simulink model "SlidingModeObserverTest"  (R2026b)
settings: Solver=FixedStepDiscrete  StopTime=smoTestCfg.Duration  FixedStep=smoCfg.Ts
PostLoadFcn:
  | addpath(fullfile(fileparts(get_param(bdroot,'FileName')),'..','build_process'));initialize_smo_test(bdroot);
model workspace (MAT data in the model file):
  pllCfg.Ts = 5e-05
  pllCfg.NaturalFrequency = 40
  pllCfg.Damping = 0.707
  pllCfg.Kp = 355.376960974
  pllCfg.Ki = 63165.468167
  pllCfg.Kaw = 502.654824574
  pllCfg.OmegaMax = 1500
  pllCfg.MinMagnitude = 1
  pllCfg.LockError = 0.12
  pllCfg.LockSamples = 100
  pllCfg.Theta0 = 0
  pllCfg.Omega0 = 0
  smoCfg.Ts = 5e-05
  smoCfg.Rs = 0.5
  smoCfg.L = 0.001
  smoCfg.Flux = 0.035
  smoCfg.PolePairs = 4
  smoCfg.SlidingGain = 30
  smoCfg.Boundary = 1
  smoCfg.FilterHz = 600
  smoCfg.MinEmf = 1
  smoCfg.MinOmega = 30
  smoCfg.Compensate = 1
  smoCfg.A = 0.975309912028
  smoCfg.B = 0.0493801759433
  smoCfg.FilterA = 0.828204181307
  smoCfg.BoundaryPole = -0.506095366272
  smoTestCfg.Duration = 0.3
  smoTestCfg.ElectricalSpeed = 200
  smoTestCfg.InitialAngle = 0.4
  smoTestCfg.Iq = 2
  testStim.time = [0 5e-05 0.0001 0.00015 0.0002 0.00025 0.0003 0.00035 0.0004 0.00045 0.0005 0.00055 ... (6001 elements, 6001x1)]
  testStim.signals.values = [-3.48377113607 -3.555722953 -3.6273192006 -3.6985527193 -3.76941638582 -3.83990311383 -3.91000585473 -3.97971759831 -4.04903137344 -4.11794024881 -4.18643733359 -4.25451577812 ... (54009 elements, 6001x9)]
  testStim.signals.dimensions = 9
libraries: SlidingModeObserver x1
settings Model: Creator=24322  LastModifiedBy=24322

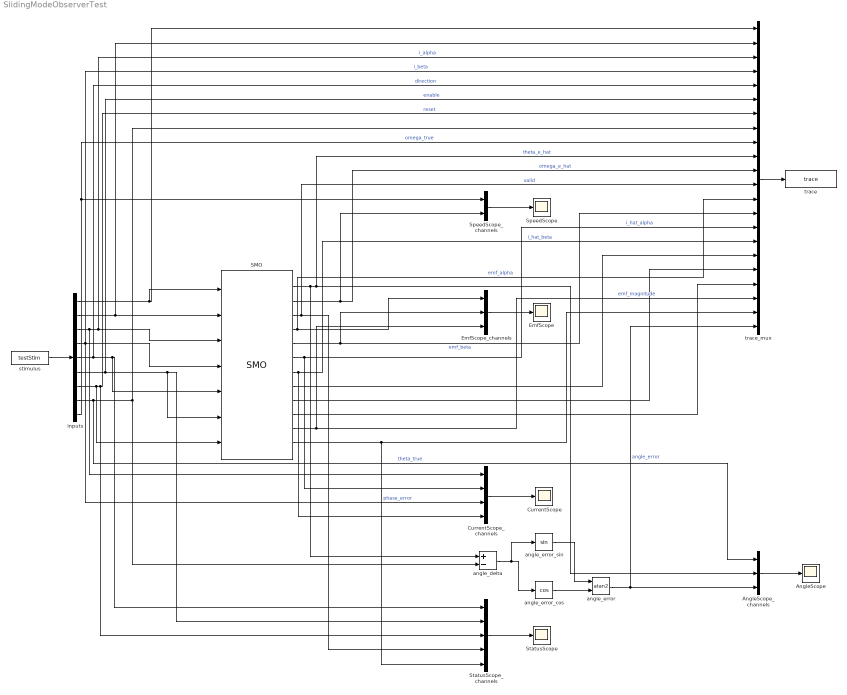
== system SlidingModeObserverTest ==
  AngleScope : Scope
  AngleScope_channels : Mux  Inputs=3
  CurrentScope : Scope
  CurrentScope_channels : Mux
  EmfScope : Scope
  EmfScope_channels : Mux  Inputs=3
  SMO : SlidingModeObserver/SMO  SystemSampleTime=-1  VariantActivationTime=update diagram  EmptyChoice=off  PassThrough=off  PassThroughVariantControl=(default)  EmptyChoiceVariantControl=(default)  AllowFlexibleInterface=on  Latency=0  AutoFrameSizeCalculation=off
  SpeedScope : Scope
  SpeedScope_channels : Mux  Inputs=2
  StatusScope : Scope
  StatusScope_channels : Mux  Inputs=5
  angle_delta : Sum  Inputs=+-
  angle_error : Trigonometry  Operator=atan2
  angle_error_cos : Trigonometry  Operator=cos
  angle_error_sin : Trigonometry
  inputs : Demux  Outputs=9
  stimulus : FromWorkspace  VariableName=testStim  SampleTime=smoCfg.Ts  Interpolate=off  OutputAfterFinalValue=Holding final value
  trace : ToWorkspace  VariableName=trace  SaveFormat=Structure With Time  SampleTime=-1
  trace_mux : Mux  Inputs=22
  wires:
  StatusScope_channels/1 -> StatusScope/1
  CurrentScope_channels/1 -> CurrentScope/1
  EmfScope_channels/1 -> EmfScope/1
  SpeedScope_channels/1 -> SpeedScope/1
  AngleScope_channels/1 -> AngleScope/1
  trace_mux/1 -> trace/1
  angle_error/1 -> trace_mux/22, AngleScope_channels/3  "angle_error"
  angle_delta/1 -> angle_error_sin/1, angle_error_cos/1
  SMO/12 -> trace_mux/21, StatusScope_channels/5  "phase_error"
  SMO/11 -> trace_mux/20, EmfScope_channels/3  "emf_magnitude"
  SMO/10 -> trace_mux/19
  SMO/9 -> trace_mux/18
  SMO/8 -> trace_mux/17
  SMO/7 -> trace_mux/16, CurrentScope_channels/4  "i_hat_beta"
  SMO/6 -> trace_mux/15, CurrentScope_channels/2  "i_hat_alpha"
  SMO/5 -> trace_mux/14, EmfScope_channels/2  "emf_beta"
  SMO/4 -> trace_mux/13, EmfScope_channels/1  "emf_alpha"
  SMO/3 -> trace_mux/12, StatusScope_channels/4  "valid"
  SMO/2 -> trace_mux/11, SpeedScope_channels/2  "omega_e_hat"
  SMO/1 -> trace_mux/10, AngleScope_channels/2, angle_delta/1  "theta_e_hat"
  inputs/9 -> trace_mux/9, SpeedScope_channels/1  "omega_true"
  inputs/8 -> trace_mux/8, angle_delta/2, AngleScope_channels/1  "theta_true"
  inputs/7 -> StatusScope_channels/3, trace_mux/7, SMO/7  "reset"
  inputs/6 -> StatusScope_channels/2, SMO/6, trace_mux/6  "enable"
  inputs/5 -> SMO/5, StatusScope_channels/1, trace_mux/5  "direction"
  inputs/4 -> CurrentScope_channels/3, SMO/4, trace_mux/4  "i_beta"
  inputs/3 -> SMO/3, trace_mux/3, CurrentScope_channels/1  "i_alpha"
  inputs/2 -> SMO/2, trace_mux/2
  inputs/1 -> SMO/1, trace_mux/1
  stimulus/1 -> inputs/1
  angle_error_cos/1 -> angle_error/2
  angle_error_sin/1 -> angle_error/1
